simulink model "lateral_bicycle"  (R2026b)
settings: Solver=FixedStepDiscrete  StartTime=0  StopTime=12  FixedStep=0.01
model workspace (MAT data in the model file):
  Ad = [0.947491632785  -0.17851011045  0  0; 0.00603414457859  0.937434725154  0  0; 3.07725423377e-05  0.00968478875686  1  0; 0.00973814804876  6.8551915025e-05  0.2  1]
  Bd = [0.484299796034; 0.373537090522; 0.00188502467186; 0.00262819892682]
  K = [0.0334182202152 0.234824970762 2.07479779913 0.157430096866]
  Ts = 0.01
  delta_increment = 0.00523598775598
  delta_limit = 0.0872664625997
  ff_input = [0 0.01 0.02 0.03 0.04 0.05 0.06 0.07 0.08 0.09 0.1 0.11 ... (2402 elements, 1201x2)]
  open_input = [0 0.01 0.02 0.03 0.04 0.05 0.06 0.07 0.08 0.09 0.1 0.11 ... (2402 elements, 1201x2)]
  ref_input = [0 0.01 0.02 0.03 0.04 0.05 0.06 0.07 0.08 0.09 0.1 0.11 ... (6005 elements, 1201x5)]
  tracking_enabled = 1
  x0 = [0; 0; 0; 0]
settings Model: Creator=volkanakyazici  LastModifiedBy=volkanakyazici

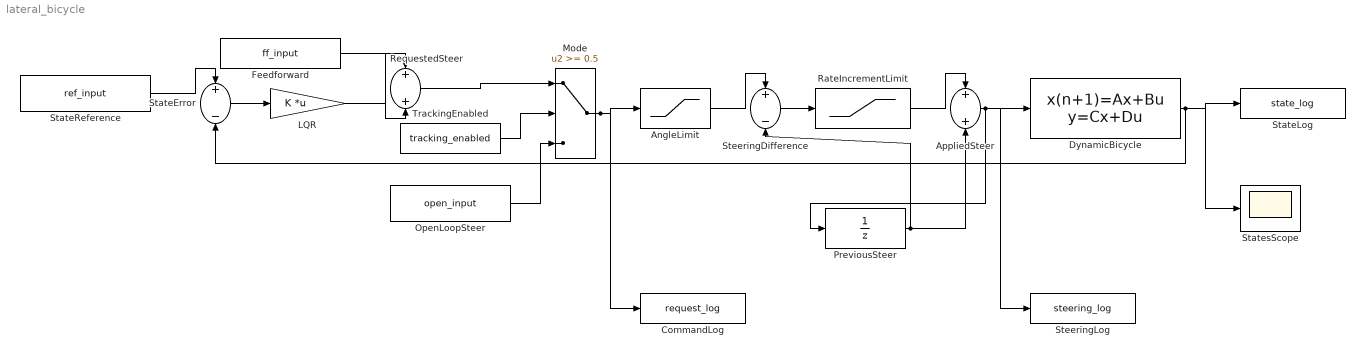
== system lateral_bicycle ==
  AngleLimit : Saturate  UpperLimit=delta_limit  LowerLimit=-delta_limit
  AppliedSteer : Sum
  CommandLog : ToWorkspace  VariableName=request_log  SaveFormat=Timeseries  SampleTime=Ts
  DynamicBicycle : DiscreteStateSpace  A=Ad  B=Bd  C=eye(4)  D=zeros(4,1)  InitialCondition=x0  SampleTime=Ts
  Feedforward : FromWorkspace  VariableName=ff_input  SampleTime=Ts  Interpolate=off  OutputAfterFinalValue=Holding final value
  LQR : Gain  Gain=K  Multiplication=Matrix(K*u) (u vector)
  Mode : Switch  Threshold=0.5  SaturateOnIntegerOverflow=off  InputSameDT=off
  OpenLoopSteer : FromWorkspace  VariableName=open_input  SampleTime=Ts  Interpolate=off  OutputAfterFinalValue=Holding final value
  PreviousSteer : UnitDelay  SampleTime=Ts
  RateIncrementLimit : Saturate  UpperLimit=delta_increment  LowerLimit=-delta_increment
  RequestedSteer : Sum
  StateError : Sum  Inputs=+-
  StateLog : ToWorkspace  VariableName=state_log  SaveFormat=Timeseries  SampleTime=Ts
  StateReference : FromWorkspace  VariableName=ref_input  SampleTime=Ts  Interpolate=off  OutputAfterFinalValue=Holding final value
  StatesScope : Scope
  SteeringDifference : Sum  Inputs=+-
  SteeringLog : ToWorkspace  VariableName=steering_log  SaveFormat=Timeseries  SampleTime=Ts
  TrackingEnabled : Constant  Value=tracking_enabled
  wires:
  StateReference/1 -> StateError/1
  DynamicBicycle/1 -> StateError/2, StateLog/1, StatesScope/1
  StateError/1 -> LQR/1
  LQR/1 -> RequestedSteer/1
  Feedforward/1 -> RequestedSteer/2
  RequestedSteer/1 -> Mode/1
  TrackingEnabled/1 -> Mode/2
  OpenLoopSteer/1 -> Mode/3
  Mode/1 -> AngleLimit/1, CommandLog/1
  AngleLimit/1 -> SteeringDifference/1
  PreviousSteer/1 -> SteeringDifference/2, AppliedSteer/2
  SteeringDifference/1 -> RateIncrementLimit/1
  RateIncrementLimit/1 -> AppliedSteer/1
  AppliedSteer/1 -> PreviousSteer/1, DynamicBicycle/1, SteeringLog/1
